simulink model "rc_circuit_calculation"  (R2026a)
settings: Solver=VariableStepAuto  StopTime=1e-3
settings Model: Creator=HAKAN SARI  LastModifiedBy=HAKAN SARI

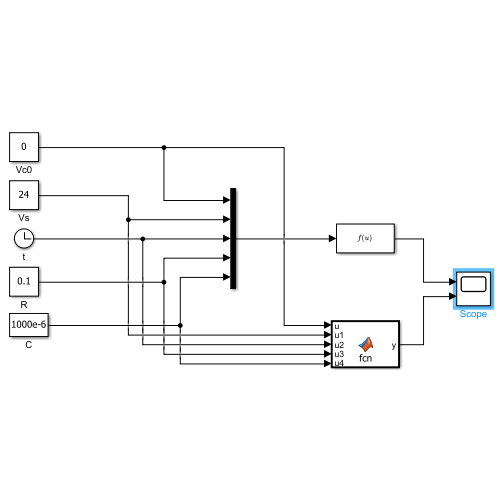
[thumbnail: Simulink's stored preview of the top-level diagram]
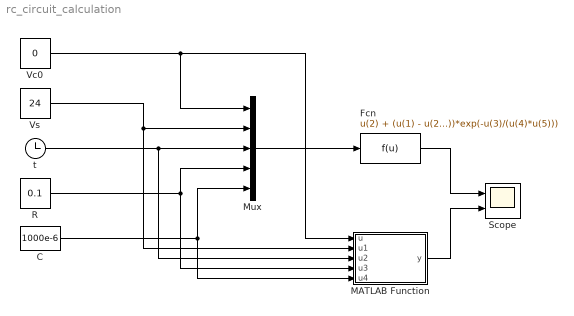
== system rc_circuit_calculation ==
  C : Constant  Value=1000e-6
  Fcn : Fcn  Expr=u(2) + (u(1) - u(2))*exp(-u(3)/(u(4)*u(5)))
  MATLAB Function : MATLAB Function  TreatAsAtomicUnit=on
  Mux : Mux  Inputs=5
  R : Constant  Value=0.1
  Scope : Scope  NumInputPorts=2
      settings: ActiveDisplayYMinimum=-3.4070121951219541  ActiveDisplayYMaximum=28.092987804878053
  Vc0 : Constant  Value=0
  Vs : Constant  Value=24
  t : Clock
  wires:
  Mux/1 -> Fcn/1
  Vc0/1 -> MATLAB Function/1(u), Mux/1
  Vs/1 -> MATLAB Function/2(u1), Mux/2
  t/1 -> MATLAB Function/3(u2), Mux/3
  R/1 -> MATLAB Function/4(u3), Mux/4
  C/1 -> MATLAB Function/5(u4), Mux/5
  Fcn/1 -> Scope/1
  MATLAB Function/1(y) -> Scope/2

== matlab function rc_circuit_calculation/MATLAB Function ==
  data: u input; y output; u1 input; u2 input; u3 input; u4 input
function y = fcn(u, u1, u2, u3, u4)

y = u1+(u-u1)*exp(-u2/(u3*u4));
